simulink model "Chap4_4a"  (R2020b)
settings: Solver=VariableStepAuto  StartTime=0.0  StopTime=10.0  RelTol=1e-3
StopFcn:
  | clc;
  | clear all;
  | close all;
  | dat=load('Data.mat','ans');
  | figure
  | plot(dat.ans.time,dat.ans.data(:,1),'-.')
  | legend('y(t)')
  | title('Response of Open System')
settings Model: Creator=yiyon  LastModifiedBy=yiyon

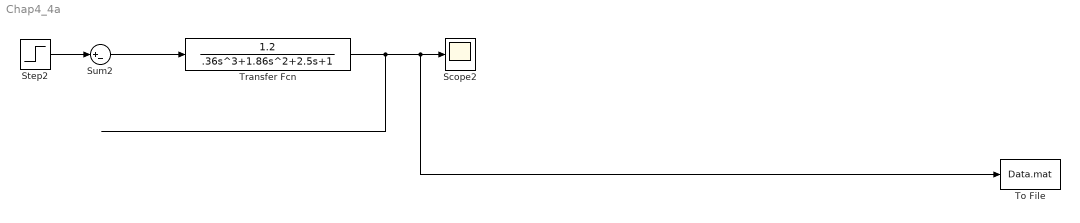
== system Chap4_4a ==
  Scope2 : Scope
  Step2 : Step  Time=0
  Sum2 : Sum  Inputs=|+-
  To File : ToFile  Filename=Data.mat  SaveFormat=Timeseries
  Transfer Fcn : TransferFcn  Numerator=[1.2]  Denominator="[.36  1.86  2.5 1]"
  wires:
  Sum2/1 -> Transfer Fcn/1
  Step2/1 -> Sum2/1
  Transfer Fcn/1 -> To File/1, Scope2/1
